simulink model "StarshipSystemModel"  (R2025b)
settings: Solver=VariableStepAuto  StartTime=0.0  StopTime=10.0  RelTol=1e-3
model workspace (MAT data in the model file):
  ActiveGNCMode : Simulink.Bus (value not decoded)
  AerodynamicControlCommand : Simulink.Bus (value not decoded)
  AerodynamicLoad : Simulink.Bus (value not decoded)
  AggregatedStream : Simulink.Bus (value not decoded)
  AllocatedEffectorDemand : Simulink.Bus (value not decoded)
  AttitudeControlDemand : Simulink.Bus (value not decoded)
  AttitudeGuidanceCommand : Simulink.Bus (value not decoded)
  AttitudeRateState : Simulink.Bus (value not decoded)
  AutogenousPressurantGas : Simulink.ConnectionBus (value not decoded)
  CandidateFaultIndication : Simulink.Bus (value not decoded)
  CombustionGasFeed : Simulink.ConnectionBus (value not decoded)
  CommandPathHealth : Simulink.Bus (value not decoded)
  ControlMode : Simulink.ValueType (value not decoded)
  DownlinkSignal : Simulink.Bus (value not decoded)
  ElectricalPower : Simulink.ConnectionBus (value not decoded)
  EngineTelemetry : Simulink.Bus (value not decoded)
  ExecutionContext : Simulink.Bus (value not decoded)
  FaultDiagnosisResult : Simulink.Bus (value not decoded)
  GNCDataContext : Simulink.Bus (value not decoded)
  GNCHealthState : Simulink.Bus (value not decoded)
  GNCStateEstimate : Simulink.Bus (value not decoded)
  GimbalAngle : Simulink.ValueType (value not decoded)
  GimbalMotion : Simulink.ConnectionBus (value not decoded)
  GroundCheckoutLink : Simulink.Bus (value not decoded)
  GroundPressurantSupply : Simulink.ConnectionBus (value not decoded)
  GuidanceConstraints : Simulink.Bus (value not decoded)
  GuidanceMode : Simulink.ValueType (value not decoded)
  LinkHealth : Simulink.Bus (value not decoded)
  LiquidPropellantFeed : Simulink.ConnectionBus (value not decoded)
  MechanicalMotion : Simulink.ConnectionBus (value not decoded)
  MechanismPosition : Simulink.Bus (value not decoded)
  ModeTransitionContext : Simulink.Bus (value not decoded)
  NavigationAidingData : Simulink.Bus (value not decoded)
  NavigationEstimate : Simulink.Bus (value not decoded)
  NavigationHealthStatus : Simulink.Bus (value not decoded)
  NavigationMeasurementSet : Simulink.Bus (value not decoded)
  PercentThrottle : Simulink.ValueType (value not decoded)
  PneumaticActuationGas : Simulink.ConnectionBus (value not decoded)
  PowerConversionStatus : Simulink.Bus (value not decoded)
  PowerDistributionStatus : Simulink.Bus (value not decoded)
  PowerHealthStatus : Simulink.Bus (value not decoded)
  PowerManagementCommand : Simulink.Bus (value not decoded)
  PowerStorageStatus : Simulink.Bus (value not decoded)
  ProtectedThermalState : Simulink.Bus (value not decoded)
  ProtectionIsolationStatus : Simulink.Bus (value not decoded)
  PurgeGasSupply : Simulink.ConnectionBus (value not decoded)
  RCSPulseCommand : Simulink.Bus (value not decoded)
  RCSTelemetry : Simulink.Bus (value not decoded)
  RFFeed : Simulink.ConnectionBus (value not decoded)
  RecoveryMechanismCommand : Simulink.Bus (value not decoded)
  RollThrottleBias : Simulink.ValueType (value not decoded)
  SafetyOverride : Simulink.ValueType (value not decoded)
  SafetyStateStatus : Simulink.Bus (value not decoded)
  ShapedControlDemand : Simulink.Bus (value not decoded)
  SpinStartIgniterGas : Simulink.ConnectionBus (value not decoded)
  StageMechanicalBoundary : Simulink.ConnectionBus (value not decoded)
  StructuralLoad : Simulink.ConnectionBus (value not decoded)
  StructureHealthStatus : Simulink.Bus (value not decoded)
  SubsystemHealthEvidence : Simulink.Bus (value not decoded)
  SubsystemStatusTelemetry : Simulink.Bus (value not decoded)
  TankTelemetry : Simulink.Bus (value not decoded)
  ThermalMonitoringCommand : Simulink.Bus (value not decoded)
  ThermalNetwork : Simulink.ConnectionBus (value not decoded)
  ThrustLoad : Simulink.ConnectionBus (value not decoded)
  TrajectoryGuidanceCommand : Simulink.Bus (value not decoded)
  TrajectoryReference : Simulink.Bus (value not decoded)
  TranslationalControlDemand : Simulink.Bus (value not decoded)
  TranslationalState : Simulink.Bus (value not decoded)
  UplinkSignal : Simulink.Bus (value not decoded)
  ValidatedControlDemand : Simulink.Bus (value not decoded)
  ValveCommand : Simulink.ValueType (value not decoded)
  VehicleStructureState : Simulink.Bus (value not decoded)
  VerifiedCommand : Simulink.Bus (value not decoded)
  VideoStream : Simulink.Bus (value not decoded)
undefined symbols (not defined in the file): ACR, ACT, ASM, ATM, BCR, BDQ, BDR, BDX, BEC, BFC, BHV, BIP, BLM, BNZ, BPI, BPR, BPV, BRX, BSM, BTA, BTP, BVC, BVE, BVV, CAA, CAM, CAS, CAT, CLM, COM, CRS, CTL, CTR, DAQ, ESC, EXT, FCR, FDB, FDE, FEX, FHI, FHM, FIC, FIS, FMG, FSC, GAP, GCM, GMD, GNC, GND, GPH, GTR, HDN, HIA, HSI, IF, INT, LOC, NAI ... (+45)
(part 4 of 8)

== system StarshipSystemModel/Starship/Power & Electrical Energy/Power Management & Monitoring ==
  Bus Element In4 : Inport  PortName=IF-BIP-PIS-01
  Bus Element In2 : Inport  Port=2  PortName=IF-PCM-PSM-01
  Bus Element In1 : Inport  Port=3  PortName=IF-BSM-PSM-01
  Bus Element In3 : Inport  Port=4  PortName=IF-HDN-PSM-01
  Bus Element In5 : Inport  Port=5  PortName=IF-HSI-PIS-01
  Bus Element In6 : Inport  Port=6  PortName=IF-BPI-PIS-01
  Power Management Coordinator : Subsystem
      settings: PortSchema="{\"entries\":[{\"content\":{\"headerSize\":26,\"margin\":15,\"minimumSpacing\":25,\"sides\":[{\"content\":{\"connectorIds\":[\"In1\"]},\"type\":\"ConnectorPlacement.EquallySpacedRectSide\",\"uuid\":\"e231466c-79f3-4a10-9258-08b328dbb315\"},{\"content\":{\"connectorIds\":[\"Out1\",\"Out2\",\"Out3\"],\"side\":\"RIGHT\"},\"type\":\"ConnectorPlacement.EquallySpacedRectSide\",\"uuid\":\"d7277c0a-5b77-426a-ad5b-7f06851f857a\"},{\"content\":{\"side\":\"TOP\"},\"type\":\"ConnectorPlacement.EquallySpacedRectSide\",\"uuid\":\"72d60576-32e4-4fd9-b552-a617024da2ce\"}]},\"type\":\"ConnectorPlacement.EquallySpacedConnector\",\"uuid\":\"6309e805-37c0-4868-97b0-5f8fd0bed587\"}],\"packageUris\":[\"http://schema.mathworks.com/mf0/Connector/R2020b\"],\"version\":\"1.0\"}"
  Power State Monitor : Subsystem
      settings: PortSchema="{\"entries\":[{\"content\":{\"headerSize\":26,\"margin\":15,\"minimumSpacing\":25,\"sides\":[{\"content\":{\"connectorIds\":[\"In2\",\"In3\",\"In1\"]},\"type\":\"ConnectorPlacement.EquallySpacedRectSide\",\"uuid\":\"e231466c-79f3-4a10-9258-08b328dbb315\"},{\"content\":{\"connectorIds\":[\"Out1\"],\"side\":\"RIGHT\"},\"type\":\"ConnectorPlacement.EquallySpacedRectSide\",\"uuid\":\"d7277c0a-5b77-426a-ad5b-7f06851f857a\"},{\"content\":{\"side\":\"TOP\"},\"type\":\"ConnectorPlacement.EquallySpacedRectSide\",\"uuid\":\"72d60576-32e4-4fd9-b552-a617024da2ce\"},{\"content\":{\"side\":\"BOTTOM\"},\"type\":\"ConnectorPlacement.EquallySpacedRectSide\",\"uuid\":\"b6db3a75-7a81-4eda-8d8a-fe1c64e0826f\"}]},\"type\":\"ConnectorPlacement.EquallySpacedConnector\",\"uuid\":\"6309e805-37c0-4868-97b0-5f8fd0bed587\"}],\"packageUris\":[\"http://schema.mathworks.com/mf0/Connector/R2020b\"],\"version\":\"1.0\"}"
  Protection / Isolation Status : Subsystem
      settings: PortSchema="{\"entries\":[{\"content\":{\"headerSize\":26,\"margin\":15,\"minimumSpacing\":25,\"sides\":[{\"content\":{\"connectorIds\":[\"In1\",\"In2\",\"In3\"]},\"type\":\"ConnectorPlacement.EquallySpacedRectSide\",\"uuid\":\"e231466c-79f3-4a10-9258-08b328dbb315\"},{\"content\":{\"side\":\"RIGHT\"},\"type\":\"ConnectorPlacement.EquallySpacedRectSide\",\"uuid\":\"d7277c0a-5b77-426a-ad5b-7f06851f857a\"},{\"content\":{\"side\":\"TOP\"},\"type\":\"ConnectorPlacement.EquallySpacedRectSide\",\"uuid\":\"72d60576-32e4-4fd9-b552-a617024da2ce\"}]},\"type\":\"ConnectorPlacement.EquallySpacedConnector\",\"uuid\":\"6309e805-37c0-4868-97b0-5f8fd0bed587\"}],\"packageUris\":[\"http://schema.mathworks.com/mf0/Connector/R2020b\"],\"version\":\"1.0\"}"
  Bus Element Out1 : Outport  PortName=IF-PMC-BIP-01
  Bus Element Out2 : Outport  Port=2  PortName=IF-PMC-HSI-01
  Bus Element Out3 : Outport  Port=3  PortName=IF-PMM-SAF-01
  wires:
  Bus Element In3/1 -> Power State Monitor/1(IF-HDN-PSM-01)
  Bus Element In5/1 -> Protection / Isolation Status/2(IF-HSI-PIS-01)
  Bus Element In1/1 -> Power State Monitor/3(IF-BSM-PSM-01)
  Bus Element In6/1 -> Protection / Isolation Status/3(IF-BPI-PIS-01)
  Bus Element In2/1 -> Power State Monitor/2(IF-PCM-PSM-01)
  Bus Element In4/1 -> Protection / Isolation Status/1(IF-BIP-PIS-01)
  Power State Monitor/1(IF-PSM-PMC-01) -> Power Management Coordinator/1(IF-PSM-PMC-01)
  Power Management Coordinator/1(IF-PMC-BIP-01) -> Bus Element Out1/1
  Power Management Coordinator/2(IF-PMC-HSI-01) -> Bus Element Out2/1
  Power Management Coordinator/3(IF-PMM-SAF-01) -> Bus Element Out3/1

== system StarshipSystemModel/Starship/Propellent system/Booster propellant System ==
  Bus Element In1 : Inport  PortName=IF-GNC-BFC-01
  Bus Element In2 : Inport  Port=2  PortName=IF-GNC-BPR-01
  Booster propellant tanks : Subsystem
      settings: PortSchema="{\"entries\":[{\"content\":{\"headerSize\":26,\"margin\":15,\"minimumSpacing\":25,\"sides\":[{\"content\":{\"connectorIds\":[\"LConn2\",\"LConn3\",\"LConn4\",\"LConn5\"]},\"type\":\"ConnectorPlacement.EquallySpacedRectSide\",\"uuid\":\"fbe4f8e6-132c-4a0c-8c4c-52d0209da778\"},{\"content\":{\"connectorIds\":[\"LConn1\",\"RConn1\",\"RConn2\",\"RConn3\",\"RConn4\",\"RConn5\"],\"side\":\"RIGHT\"},\"type\":\"ConnectorPlacement.EquallySpacedRectSide\",\"uuid\":\"bbe80fa3-b8e3-44c5-9574-5758a55378fd\"},{\"content\":{\"side\":\"TOP\"},\"type\":\"ConnectorPlacement.EquallySpacedRectSide\",\"uuid\":\"410005e2-e10b-4d3e-a617-d51b1ea5de7e\"}]},\"type\":\"ConnectorPlacement.EquallySpacedConnector\",\"uuid\":\"b66a347a-e5b4-46b1-8a3f-28cf70f30a27\"}],\"packageUris\":[\"http://schema.mathworks.com/mf0/Connector/R2020b\"],\"version\":\"1.0\"}"
  Feed & distribution : Subsystem
      settings: PortSchema="{\"entries\":[{\"content\":{\"headerSize\":26,\"margin\":15,\"minimumSpacing\":25,\"sides\":[{\"content\":{\"connectorIds\":[\"LConn1\",\"LConn2\",\"LConn3\",\"LConn4\",\"LConn5\",\"In1\",\"LConn6\"]},\"type\":\"ConnectorPlacement.EquallySpacedRectSide\",\"uuid\":\"fbe4f8e6-132c-4a0c-8c4c-52d0209da778\"},{\"content\":{\"connectorIds\":[\"RConn1\"],\"side\":\"RIGHT\"},\"type\":\"ConnectorPlacement.EquallySpacedRectSide\",\"uuid\":\"bbe80fa3-b8e3-44c5-9574-5758a55378fd\"},{\"content\":{\"side\":\"TOP\"},\"type\":\"ConnectorPlacement.EquallySpacedRectSide\",\"uuid\":\"410005e2-e10b-4d3e-a617-d51b1ea5de7e\"}]},\"type\":\"ConnectorPlacement.EquallySpacedConnector\",\"uuid\":\"b66a347a-e5b4-46b1-8a3f-28cf70f30a27\"}],\"packageUris\":[\"http://schema.mathworks.com/mf0/Connector/R2020b\"],\"version\":\"1.0\"}"
  Ground propellant interface : Subsystem
      settings: PortSchema="{\"entries\":[{\"content\":{\"headerSize\":26,\"margin\":15,\"minimumSpacing\":25,\"sides\":[{\"content\":{\"connectorIds\":[\"LConn1\",\"LConn2\",\"LConn3\"]},\"type\":\"ConnectorPlacement.EquallySpacedRectSide\",\"uuid\":\"fbe4f8e6-132c-4a0c-8c4c-52d0209da778\"},{\"content\":{\"connectorIds\":[\"RConn1\",\"RConn5\",\"RConn3\",\"RConn2\",\"RConn4\"],\"side\":\"RIGHT\"},\"type\":\"ConnectorPlacement.EquallySpacedRectSide\",\"uuid\":\"bbe80fa3-b8e3-44c5-9574-5758a55378fd\"},{\"content\":{\"side\":\"TOP\"},\"type\":\"ConnectorPlacement.EquallySpacedRectSide\",\"uuid\":\"410005e2-e10b-4d3e-a617-d51b1ea5de7e\"}]},\"type\":\"ConnectorPlacement.EquallySpacedConnector\",\"uuid\":\"b66a347a-e5b4-46b1-8a3f-28cf70f30a27\"}],\"packageUris\":[\"http://schema.mathworks.com/mf0/Connector/R2020b\"],\"version\":\"1.0\"}"
  "Pressurization, purge & venting" : Subsystem
      settings: PortSchema="{\"entries\":[{\"content\":{\"headerSize\":26,\"margin\":15,\"minimumSpacing\":25,\"sides\":[{\"content\":{\"connectorIds\":[\"LConn1\",\"LConn2\",\"LConn3\",\"LConn4\",\"LConn5\",\"LConn6\",\"In1\",\"LConn7\"]},\"type\":\"ConnectorPlacement.EquallySpacedRectSide\",\"uuid\":\"fbe4f8e6-132c-4a0c-8c4c-52d0209da778\"},{\"content\":{\"connectorIds\":[\"RConn1\",\"Out1\",\"RConn2\",\"RConn3\",\"RConn4\",\"RConn5\",\"Out2\",\"RConn6\"],\"side\":\"RIGHT\"},\"type\":\"ConnectorPlacement.EquallySpacedRectSide\",\"uuid\":\"bbe80fa3-b8e3-44c5-9574-5758a55378fd\"},{\"content\":{\"side\":\"TOP\"},\"type\":\"ConnectorPlacement.EquallySpacedRectSide\",\"uuid\":\"410005e2-e10b-4d3e-a617-d51b1ea5de7e\"}]},\"type\":\"ConnectorPlacement.EquallySpacedConnector\",\"uuid\":\"b66a347a-e5b4-46b1-8a3f-28cf70f30a27\"}],\"packageUris\":[\"http://schema.mathworks.com/mf0/Connector/R2020b\"],\"version\":\"1.0\"}"
  IF-BDM-BTP-01 : PMIOPort  Side=Right  ConnectionType=Bus: LiquidPropellantFeed
  IF-BSG-BIG-01 : PMIOPort  Port=2  Side=Right  ConnectionType=Bus: SpinStartIgniterGas
  IF-BNG-BVC-01 : PMIOPort  Port=3  Side=Right  ConnectionType=Bus: PneumaticActuationGas
  IF-BOT-PRS-01 : PMIOPort  Port=4  Side=Left  ConnectionType=Bus: StructuralLoad
  IF-BTP-BPR-01 : PMIOPort  Port=5  Side=Left  ConnectionType=Bus: AutogenousPressurantGas
  "IF-GND-BLQ-01\t" : PMIOPort  Port=6  Side=Left
  "IF-GND-BCQ-01\t" : PMIOPort  Port=7  Side=Left
  IF-PWR-BFC-01 : PMIOPort  Port=8  Side=Left  ConnectionType=Bus: ElectricalPower
  IF-PWR-BPR-01 : PMIOPort  Port=9  Side=Left  ConnectionType=Bus: ElectricalPower
  IF-GND-BPQ-01 : PMIOPort  Port=10  Side=Left  ConnectionType=Bus: GroundPressurantSupply
  Bus Element Out1 : Outport  PortName=IF-BPR-SAF-01
  Bus Element Out2 : Outport  Port=2  PortName=IF-BPR-BTA-01
  wires:
  Bus Element In2/1 -> "Pressurization, purge & venting"/1(IF-GNC-BPR-01)
  "Pressurization, purge & venting"/2(IF-BPR-SAF-01) -> Bus Element Out1/1
  "Pressurization, purge & venting"/1(IF-BPR-BTA-01) -> Bus Element Out2/1
  Bus Element In1/1 -> Feed & distribution/1(IF-GNC-BFC-01)
  connections:
  "IF-GND-BCQ-01\t"/RConn1 -- Ground propellant interface/LConn2
  IF-GND-BPQ-01/RConn1 -- Ground propellant interface/LConn3
  "IF-GND-BLQ-01\t"/RConn1 -- Ground propellant interface/LConn1
  Ground propellant interface/RConn2 -- "Pressurization, purge & venting"/LConn3
  Ground propellant interface/RConn3 -- "Pressurization, purge & venting"/LConn2
  Ground propellant interface/RConn1 -- Booster propellant tanks/LConn2
  Ground propellant interface/RConn5 -- Booster propellant tanks/LConn4
  Ground propellant interface/RConn4 -- "Pressurization, purge & venting"/LConn1
  IF-BTP-BPR-01/RConn1 -- "Pressurization, purge & venting"/LConn4
  "Pressurization, purge & venting"/RConn1 -- IF-BSG-BIG-01/RConn1
  Feed & distribution/RConn1 -- IF-BDM-BTP-01/RConn1
  "Pressurization, purge & venting"/RConn2 -- Booster propellant tanks/LConn5
  "Pressurization, purge & venting"/RConn3 -- Feed & distribution/LConn3
  "Pressurization, purge & venting"/RConn4 -- Feed & distribution/LConn4
  "Pressurization, purge & venting"/RConn5 -- Booster propellant tanks/LConn3
  "Pressurization, purge & venting"/RConn6 -- IF-BNG-BVC-01/RConn1
  Booster propellant tanks/RConn5 -- Feed & distribution/LConn2
  Booster propellant tanks/RConn1 -- Feed & distribution/LConn1
  Booster propellant tanks/RConn2 -- Feed & distribution/LConn5
  Booster propellant tanks/RConn3 -- "Pressurization, purge & venting"/LConn6
  Booster propellant tanks/RConn4 -- "Pressurization, purge & venting"/LConn5
  IF-BOT-PRS-01/RConn1 -- Booster propellant tanks/LConn1
  IF-PWR-BFC-01/RConn1 -- Feed & distribution/LConn6
  IF-PWR-BPR-01/RConn1 -- "Pressurization, purge & venting"/LConn7

== system StarshipSystemModel/Starship/Propellent system/Ship propellant System ==
  Bus Element In1 : Inport  PortName=IF-GNC-SFC-01
  Bus Element In2 : Inport  Port=2  PortName=IF-GNC-SPR-01
  Feed & distribution : Subsystem
      settings: PortSchema="{\"entries\":[{\"content\":{\"headerSize\":26,\"margin\":15,\"minimumSpacing\":25,\"sides\":[{\"content\":{\"connectorIds\":[\"LConn1\",\"In1\",\"LConn2\",\"LConn3\",\"LConn4\",\"LConn5\",\"LConn6\",\"LConn7\"]},\"type\":\"ConnectorPlacement.EquallySpacedRectSide\",\"uuid\":\"fbe4f8e6-132c-4a0c-8c4c-52d0209da778\"},{\"content\":{\"connectorIds\":[\"RConn1\"],\"side\":\"RIGHT\"},\"type\":\"ConnectorPlacement.EquallySpacedRectSide\",\"uuid\":\"bbe80fa3-b8e3-44c5-9574-5758a55378fd\"},{\"content\":{\"side\":\"TOP\"},\"type\":\"ConnectorPlacement.EquallySpacedRectSide\",\"uuid\":\"410005e2-e10b-4d3e-a617-d51b1ea5de7e\"}]},\"type\":\"ConnectorPlacement.EquallySpacedConnector\",\"uuid\":\"b66a347a-e5b4-46b1-8a3f-28cf70f30a27\"}],\"packageUris\":[\"http://schema.mathworks.com/mf0/Connector/R2020b\"],\"version\":\"1.0\"}"
  Ground propellant interface : Subsystem
      settings: PortSchema="{\"entries\":[{\"content\":{\"headerSize\":26,\"margin\":15,\"minimumSpacing\":25,\"sides\":[{\"content\":{\"connectorIds\":[\"LConn1\",\"LConn2\",\"LConn3\"]},\"type\":\"ConnectorPlacement.EquallySpacedRectSide\",\"uuid\":\"fbe4f8e6-132c-4a0c-8c4c-52d0209da778\"},{\"content\":{\"connectorIds\":[\"RConn1\",\"RConn2\",\"RConn3\",\"RConn4\",\"RConn5\"],\"side\":\"RIGHT\"},\"type\":\"ConnectorPlacement.EquallySpacedRectSide\",\"uuid\":\"bbe80fa3-b8e3-44c5-9574-5758a55378fd\"},{\"content\":{\"side\":\"TOP\"},\"type\":\"ConnectorPlacement.EquallySpacedRectSide\",\"uuid\":\"410005e2-e10b-4d3e-a617-d51b1ea5de7e\"}]},\"type\":\"ConnectorPlacement.EquallySpacedConnector\",\"uuid\":\"b66a347a-e5b4-46b1-8a3f-28cf70f30a27\"}],\"packageUris\":[\"http://schema.mathworks.com/mf0/Connector/R2020b\"],\"version\":\"1.0\"}"
  "Pressurization, purge & venting" : Subsystem
      settings: PortSchema="{\"entries\":[{\"content\":{\"headerSize\":26,\"margin\":15,\"minimumSpacing\":25,\"sides\":[{\"content\":{\"connectorIds\":[\"LConn1\",\"LConn2\",\"LConn3\",\"LConn4\",\"LConn5\",\"LConn6\",\"In1\",\"LConn7\"]},\"type\":\"ConnectorPlacement.EquallySpacedRectSide\",\"uuid\":\"fbe4f8e6-132c-4a0c-8c4c-52d0209da778\"},{\"content\":{\"connectorIds\":[\"RConn1\",\"Out1\",\"RConn2\",\"RConn3\",\"RConn4\",\"RConn5\",\"Out2\",\"RConn6\",\"RConn7\"],\"side\":\"RIGHT\"},\"type\":\"ConnectorPlacement.EquallySpacedRectSide\",\"uuid\":\"bbe80fa3-b8e3-44c5-9574-5758a55378fd\"},{\"content\":{\"side\":\"TOP\"},\"type\":\"ConnectorPlacement.EquallySpacedRectSide\",\"uuid\":\"410005e2-e10b-4d3e-a617-d51b1ea5de7e\"}]},\"type\":\"ConnectorPlacement.EquallySpacedConnector\",\"uuid\":\"b66a347a-e5b4-46b1-8a3f-28cf70f30a27\"}],\"packageUris\":[\"http://schema.mathworks.com/mf0/Connector/R2020b\"],\"version\":\"1.0\"}"
  Ship propellant tanks : Subsystem
      settings: PortSchema="{\"entries\":[{\"content\":{\"headerSize\":26,\"margin\":15,\"minimumSpacing\":25,\"sides\":[{\"content\":{\"connectorIds\":[\"LConn2\",\"LConn3\",\"LConn4\",\"LConn5\"]},\"type\":\"ConnectorPlacement.EquallySpacedRectSide\",\"uuid\":\"fbe4f8e6-132c-4a0c-8c4c-52d0209da778\"},{\"content\":{\"connectorIds\":[\"LConn1\",\"RConn4\",\"RConn1\",\"RConn3\",\"RConn2\",\"RConn5\",\"RConn6\"],\"side\":\"RIGHT\"},\"type\":\"ConnectorPlacement.EquallySpacedRectSide\",\"uuid\":\"bbe80fa3-b8e3-44c5-9574-5758a55378fd\"},{\"content\":{\"side\":\"TOP\"},\"type\":\"ConnectorPlacement.EquallySpacedRectSide\",\"uuid\":\"410005e2-e10b-4d3e-a617-d51b1ea5de7e\"}]},\"type\":\"ConnectorPlacement.EquallySpacedConnector\",\"uuid\":\"b66a347a-e5b4-46b1-8a3f-28cf70f30a27\"}],\"packageUris\":[\"http://schema.mathworks.com/mf0/Connector/R2020b\"],\"version\":\"1.0\"}"
  IF-PWR-SPR-01 : PMIOPort  Side=Right  ConnectionType=Bus: ElectricalPower
  IF-SSG-SIG-01 : PMIOPort  Port=2  Side=Right  ConnectionType=Bus: SpinStartIgniterGas
  IF-SNG-SVC-01 : PMIOPort  Port=3  Side=Right  ConnectionType=Bus: PneumaticActuationGas
  IF-SPR-RVM-01 : PMIOPort  Port=4  Side=Right  ConnectionType=Bus: CombustionGasFeed
  IF-SDM-STP-01 : PMIOPort  Port=5  Side=Right  ConnectionType=Bus: LiquidPropellantFeed
  IF-SOT-PRS-01 : PMIOPort  Port=6  Side=Left  ConnectionType=Bus: StructuralLoad
  IF-STP-SPR-01 : PMIOPort  Port=7  Side=Left  ConnectionType=Bus: AutogenousPressurantGas
  IF-GND-SLQ-01 : PMIOPort  Port=8  Side=Left
  IF-GND-SCQ-01 : PMIOPort  Port=9  Side=Left
  IF-PWR-SFC-01 : PMIOPort  Port=10  Side=Left  ConnectionType=Bus: ElectricalPower
  IF-GND-SPQ-01 : PMIOPort  Port=11  Side=Left  ConnectionType=Bus: GroundPressurantSupply
  Bus Element Out1 : Outport  PortName=IF-SPR-SAF-01
  Bus Element Out2 : Outport  Port=2  PortName=IF-SPR-STA-01
  wires:
  Bus Element In2/1 -> "Pressurization, purge & venting"/1(IF-GNC-SPR-01)
  Bus Element In1/1 -> Feed & distribution/1(IF-GNC-SFC-01)
  "Pressurization, purge & venting"/2(IF-SPR-STA-01) -> Bus Element Out2/1
  "Pressurization, purge & venting"/1(IF-SPR-SAF-01) -> Bus Element Out1/1
  connections:
  IF-GND-SPQ-01/RConn1 -- Ground propellant interface/LConn3
  IF-GND-SCQ-01/RConn1 -- Ground propellant interface/LConn2
  IF-GND-SLQ-01/RConn1 -- Ground propellant interface/LConn1
  Ground propellant interface/RConn5 -- Ship propellant tanks/LConn4
  Ground propellant interface/RConn4 -- "Pressurization, purge & venting"/LConn6
  Ground propellant interface/RConn3 -- "Pressurization, purge & venting"/LConn5
  Ground propellant interface/RConn2 -- "Pressurization, purge & venting"/LConn4
  Ground propellant interface/RConn1 -- Ship propellant tanks/LConn5
  IF-STP-SPR-01/RConn1 -- "Pressurization, purge & venting"/LConn1
  Ship propellant tanks/RConn4 -- "Pressurization, purge & venting"/LConn2
  "Pressurization, purge & venting"/RConn4 -- Feed & distribution/LConn1
  Ship propellant tanks/RConn1 -- Feed & distribution/LConn2
  "Pressurization, purge & venting"/RConn7 -- IF-SPR-RVM-01/RConn1
  Ship propellant tanks/RConn3 -- "Pressurization, purge & venting"/LConn3
  Ship propellant tanks/RConn2 -- Feed & distribution/LConn3
  "Pressurization, purge & venting"/RConn2 -- Ship propellant tanks/LConn3
  Ship propellant tanks/RConn5 -- Feed & distribution/LConn4
  Ship propellant tanks/RConn6 -- Feed & distribution/LConn5
  "Pressurization, purge & venting"/RConn5 -- Feed & distribution/LConn6
  "Pressurization, purge & venting"/RConn1 -- IF-SSG-SIG-01/RConn1
  "Pressurization, purge & venting"/RConn3 -- Ship propellant tanks/LConn2
  "Pressurization, purge & venting"/RConn6 -- IF-SNG-SVC-01/RConn1
  Feed & distribution/RConn1 -- IF-SDM-STP-01/RConn1
  IF-SOT-PRS-01/RConn1 -- Ship propellant tanks/LConn1
  IF-PWR-SFC-01/RConn1 -- Feed & distribution/LConn7
  IF-PWR-SPR-01/RConn1 -- "Pressurization, purge & venting"/LConn7

== system StarshipSystemModel/Starship/Propulsion/Booster main engines ==
  Bus Element In1 : Inport  PortName=IF-GNC-BEC-01
  Bus Element In2 : Inport  Port=2  PortName=IF-SAF-BEC-01
  "Combustion Chamber " : Subsystem
      settings: PortSchema="{\"entries\":[{\"content\":{\"headerSize\":26,\"margin\":15,\"minimumSpacing\":25,\"sides\":[{\"content\":{\"connectorIds\":[\"LConn1\"]},\"type\":\"ConnectorPlacement.EquallySpacedRectSide\",\"uuid\":\"315fc4b8-96c1-4575-a6b3-eadee3c565c5\"},{\"content\":{\"connectorIds\":[\"RConn1\"],\"side\":\"RIGHT\"},\"type\":\"ConnectorPlacement.EquallySpacedRectSide\",\"uuid\":\"3e876d4b-731c-46c4-97d4-16d95cf44eb6\"},{\"content\":{\"side\":\"TOP\"},\"type\":\"ConnectorPlacement.EquallySpacedRectSide\",\"uuid\":\"b527a8d5-4fb1-4a9d-8105-fff73624f75e\"}]},\"type\":\"ConnectorPlacement.EquallySpacedConnector\",\"uuid\":\"4da3c338-7f32-408f-a75b-02b41c006a8f\"}],\"packageUris\":[\"http://schema.mathworks.com/mf0/Connector/R2020b\"],\"version\":\"1.0\"}"
  Engine controller : Subsystem
      settings: PortSchema="{\"entries\":[{\"content\":{\"headerSize\":26,\"margin\":15,\"minimumSpacing\":25,\"sides\":[{\"content\":{\"connectorIds\":[\"LConn1\",\"In1\",\"In2\"]},\"type\":\"ConnectorPlacement.EquallySpacedRectSide\",\"uuid\":\"a24f90f9-b52e-4407-98a2-61cef3ed1001\"},{\"content\":{\"connectorIds\":[\"Out1\",\"Out2\",\"Out3\"],\"side\":\"RIGHT\"},\"type\":\"ConnectorPlacement.EquallySpacedRectSide\",\"uuid\":\"349c89d4-9966-4ad9-ba76-db4d38641e72\"},{\"content\":{\"side\":\"TOP\"},\"type\":\"ConnectorPlacement.EquallySpacedRectSide\",\"uuid\":\"c23b8a3e-5693-4bb4-96b3-90d999333c4e\"}]},\"type\":\"ConnectorPlacement.EquallySpacedConnector\",\"uuid\":\"ab682651-c32f-4460-8c4f-01dcf64563ad\"}],\"packageUris\":[\"http://schema.mathworks.com/mf0/Connector/R2020b\"],\"version\":\"1.0\"}"
  Ignition system : Subsystem
      settings: PortSchema="{\"entries\":[{\"content\":{\"headerSize\":26,\"margin\":15,\"minimumSpacing\":25,\"sides\":[{\"content\":{\"connectorIds\":[\"LConn1\"]},\"type\":\"ConnectorPlacement.EquallySpacedRectSide\",\"uuid\":\"a24f90f9-b52e-4407-98a2-61cef3ed1001\"},{\"content\":{\"connectorIds\":[\"RConn1\"],\"side\":\"RIGHT\"},\"type\":\"ConnectorPlacement.EquallySpacedRectSide\",\"uuid\":\"349c89d4-9966-4ad9-ba76-db4d38641e72\"},{\"content\":{\"side\":\"TOP\"},\"type\":\"ConnectorPlacement.EquallySpacedRectSide\",\"uuid\":\"c23b8a3e-5693-4bb4-96b3-90d999333c4e\"}]},\"type\":\"ConnectorPlacement.EquallySpacedConnector\",\"uuid\":\"ab682651-c32f-4460-8c4f-01dcf64563ad\"}],\"packageUris\":[\"http://schema.mathworks.com/mf0/Connector/R2020b\"],\"version\":\"1.0\"}"
  Mounting interface : Subsystem
      settings: PortSchema="{\"entries\":[{\"content\":{\"headerSize\":26,\"margin\":15,\"minimumSpacing\":25,\"sides\":[{\"content\":{\"connectorIds\":[\"LConn1\"]},\"type\":\"ConnectorPlacement.EquallySpacedRectSide\",\"uuid\":\"a24f90f9-b52e-4407-98a2-61cef3ed1001\"},{\"content\":{\"connectorIds\":[\"RConn1\"],\"side\":\"RIGHT\"},\"type\":\"ConnectorPlacement.EquallySpacedRectSide\",\"uuid\":\"349c89d4-9966-4ad9-ba76-db4d38641e72\"},{\"content\":{\"side\":\"TOP\"},\"type\":\"ConnectorPlacement.EquallySpacedRectSide\",\"uuid\":\"c23b8a3e-5693-4bb4-96b3-90d999333c4e\"}]},\"type\":\"ConnectorPlacement.EquallySpacedConnector\",\"uuid\":\"ab682651-c32f-4460-8c4f-01dcf64563ad\"}],\"packageUris\":[\"http://schema.mathworks.com/mf0/Connector/R2020b\"],\"version\":\"1.0\"}"
  Nozzle : Subsystem
      settings: PortSchema="{\"entries\":[{\"content\":{\"headerSize\":26,\"margin\":15,\"minimumSpacing\":25,\"sides\":[{\"content\":{\"connectorIds\":[\"LConn1\"]},\"type\":\"ConnectorPlacement.EquallySpacedRectSide\",\"uuid\":\"315fc4b8-96c1-4575-a6b3-eadee3c565c5\"},{\"content\":{\"connectorIds\":[\"Out1\"],\"side\":\"RIGHT\"},\"type\":\"ConnectorPlacement.EquallySpacedRectSide\",\"uuid\":\"3e876d4b-731c-46c4-97d4-16d95cf44eb6\"},{\"content\":{\"side\":\"TOP\"},\"type\":\"ConnectorPlacement.EquallySpacedRectSide\",\"uuid\":\"b527a8d5-4fb1-4a9d-8105-fff73624f75e\"}]},\"type\":\"ConnectorPlacement.EquallySpacedConnector\",\"uuid\":\"4da3c338-7f32-408f-a75b-02b41c006a8f\"}],\"packageUris\":[\"http://schema.mathworks.com/mf0/Connector/R2020b\"],\"version\":\"1.0\"}"
  Preburners : Subsystem
      settings: PortSchema="{\"entries\":[{\"content\":{\"headerSize\":26,\"margin\":15,\"minimumSpacing\":25,\"sides\":[{\"content\":{\"connectorIds\":[\"LConn1\",\"LConn2\"]},\"type\":\"ConnectorPlacement.EquallySpacedRectSide\",\"uuid\":\"315fc4b8-96c1-4575-a6b3-eadee3c565c5\"},{\"content\":{\"connectorIds\":[\"RConn1\"],\"side\":\"RIGHT\"},\"type\":\"ConnectorPlacement.EquallySpacedRectSide\",\"uuid\":\"3e876d4b-731c-46c4-97d4-16d95cf44eb6\"},{\"content\":{\"side\":\"TOP\"},\"type\":\"ConnectorPlacement.EquallySpacedRectSide\",\"uuid\":\"b527a8d5-4fb1-4a9d-8105-fff73624f75e\"}]},\"type\":\"ConnectorPlacement.EquallySpacedConnector\",\"uuid\":\"4da3c338-7f32-408f-a75b-02b41c006a8f\"}],\"packageUris\":[\"http://schema.mathworks.com/mf0/Connector/R2020b\"],\"version\":\"1.0\"}"
  Turbopumps : Subsystem
      settings: PortSchema="{\"entries\":[{\"content\":{\"headerSize\":26,\"margin\":15,\"minimumSpacing\":25,\"sides\":[{\"content\":{\"connectorIds\":[\"LConn1\",\"LConn2\"]},\"type\":\"ConnectorPlacement.EquallySpacedRectSide\",\"uuid\":\"315fc4b8-96c1-4575-a6b3-eadee3c565c5\"},{\"content\":{\"connectorIds\":[\"RConn1\",\"RConn2\"],\"side\":\"RIGHT\"},\"type\":\"ConnectorPlacement.EquallySpacedRectSide\",\"uuid\":\"3e876d4b-731c-46c4-97d4-16d95cf44eb6\"},{\"content\":{\"side\":\"TOP\"},\"type\":\"ConnectorPlacement.EquallySpacedRectSide\",\"uuid\":\"b527a8d5-4fb1-4a9d-8105-fff73624f75e\"}]},\"type\":\"ConnectorPlacement.EquallySpacedConnector\",\"uuid\":\"4da3c338-7f32-408f-a75b-02b41c006a8f\"}],\"packageUris\":[\"http://schema.mathworks.com/mf0/Connector/R2020b\"],\"version\":\"1.0\"}"
  Valves & control : Subsystem
      settings: PortSchema="{\"entries\":[{\"content\":{\"headerSize\":26,\"margin\":15,\"minimumSpacing\":25,\"sides\":[{\"content\":{\"connectorIds\":[\"In1\",\"LConn1\"]},\"type\":\"ConnectorPlacement.EquallySpacedRectSide\",\"uuid\":\"a24f90f9-b52e-4407-98a2-61cef3ed1001\"},{\"content\":{\"connectorIds\":[\"RConn1\"],\"side\":\"RIGHT\"},\"type\":\"ConnectorPlacement.EquallySpacedRectSide\",\"uuid\":\"349c89d4-9966-4ad9-ba76-db4d38641e72\"},{\"content\":{\"side\":\"TOP\"},\"type\":\"ConnectorPlacement.EquallySpacedRectSide\",\"uuid\":\"c23b8a3e-5693-4bb4-96b3-90d999333c4e\"}]},\"type\":\"ConnectorPlacement.EquallySpacedConnector\",\"uuid\":\"ab682651-c32f-4460-8c4f-01dcf64563ad\"}],\"packageUris\":[\"http://schema.mathworks.com/mf0/Connector/R2020b\"],\"version\":\"1.0\"}"
  IF-PWR-BEC-01 : PMIOPort  Side=Left  ConnectionType=Bus: ElectricalPower
  IF-BMT-TLI-01 : PMIOPort  Port=2  Side=Left  ConnectionType=Bus: StructuralLoad
  IF-BDM-BTP-01 : PMIOPort  Port=3  Side=Left  ConnectionType=Bus: LiquidPropellantFeed
  IF-BTP-BPR-01 : PMIOPort  Port=4  Side=Right  ConnectionType=Bus: AutogenousPressurantGas
  IF-BSG-BIG-01 : PMIOPort  Port=5  Side=Left  ConnectionType=Bus: SpinStartIgniterGas
  IF-BNG-BVC-01 : PMIOPort  Port=6  Side=Left  ConnectionType=Bus: PneumaticActuationGas
  IF-GMB-BMT-01 : PMIOPort  Port=7  Side=Left  ConnectionType=Bus: GimbalMotion
  Bus Element Out1 : Outport  PortName=IF-BEC-SAF-01
  Bus Element Out2 : Outport  Port=2  PortName=IF-BEC-BTA-01
  Bus Element Out3 : Outport  Port=3  PortName=IF-BNZ-BTP-01
  wires:
  Bus Element In2/1 -> Engine controller/2(IF-SAF-BEC-01)
  Bus Element In1/1 -> Engine controller/1(IF-GNC-BEC-01)
  Engine controller/2(IF-BEC-BTA-01) -> Bus Element Out2/1
  Engine controller/1(IF-BEC-SAF-01) -> Bus Element Out1/1
  Engine controller/3(IF-BEC-BVC-01) -> Valves & control/1(IF-BEC-BVC-01)
  Nozzle/1(IF-BNZ-BTP-01) -> Bus Element Out3/1
  connections:
  IF-BDM-BTP-01/RConn1 -- Turbopumps/LConn1
  IF-GMB-BMT-01/RConn1 -- Mounting interface/LConn1
  Preburners/RConn1 -- "Combustion Chamber "/LConn1
  Valves & control/RConn1 -- Turbopumps/LConn2
  Turbopumps/RConn2 -- Preburners/LConn1
  Ignition system/RConn1 -- Preburners/LConn2
  "Combustion Chamber "/RConn1 -- Nozzle/LConn1
  IF-BSG-BIG-01/RConn1 -- Ignition system/LConn1
  IF-BNG-BVC-01/RConn1 -- Valves & control/LConn1
  Turbopumps/RConn1 -- IF-BTP-BPR-01/RConn1
  IF-BMT-TLI-01/RConn1 -- Mounting interface/RConn1
  IF-PWR-BEC-01/RConn1 -- Engine controller/LConn1

== system StarshipSystemModel/Starship/Propulsion/Gimbal // TVC actuation ==
  Bus Element In1 : Inport  PortName=IF-GNC-TVC-01
  Gimbal bearing : Subsystem
      settings: PortSchema="{\"entries\":[{\"content\":{\"headerSize\":26,\"margin\":15,\"minimumSpacing\":25,\"sides\":[{\"content\":{\"connectorIds\":[\"LConn1\",\"LConn2\"]},\"type\":\"ConnectorPlacement.EquallySpacedRectSide\",\"uuid\":\"a24f90f9-b52e-4407-98a2-61cef3ed1001\"},{\"content\":{\"connectorIds\":[\"RConn1\",\"RConn2\"],\"side\":\"RIGHT\"},\"type\":\"ConnectorPlacement.EquallySpacedRectSide\",\"uuid\":\"349c89d4-9966-4ad9-ba76-db4d38641e72\"},{\"content\":{\"side\":\"TOP\"},\"type\":\"ConnectorPlacement.EquallySpacedRectSide\",\"uuid\":\"c23b8a3e-5693-4bb4-96b3-90d999333c4e\"}]},\"type\":\"ConnectorPlacement.EquallySpacedConnector\",\"uuid\":\"ab682651-c32f-4460-8c4f-01dcf64563ad\"}],\"packageUris\":[\"http://schema.mathworks.com/mf0/Connector/R2020b\"],\"version\":\"1.0\"}"
  Pitch actuator : Subsystem
      settings: PortSchema="{\"entries\":[{\"content\":{\"headerSize\":26,\"margin\":15,\"minimumSpacing\":25,\"sides\":[{\"content\":{\"connectorIds\":[\"In1\"]},\"type\":\"ConnectorPlacement.EquallySpacedRectSide\",\"uuid\":\"a24f90f9-b52e-4407-98a2-61cef3ed1001\"},{\"content\":{\"connectorIds\":[\"RConn1\"],\"side\":\"RIGHT\"},\"type\":\"ConnectorPlacement.EquallySpacedRectSide\",\"uuid\":\"349c89d4-9966-4ad9-ba76-db4d38641e72\"},{\"content\":{\"side\":\"TOP\"},\"type\":\"ConnectorPlacement.EquallySpacedRectSide\",\"uuid\":\"c23b8a3e-5693-4bb4-96b3-90d999333c4e\"},{\"content\":{\"side\":\"BOTTOM\"},\"type\":\"ConnectorPlacement.EquallySpacedRectSide\",\"uuid\":\"53421d2e-cd64-4a64-9551-ba2d9208335d\"}]},\"type\":\"ConnectorPlacement.EquallySpacedConnector\",\"uuid\":\"ab682651-c32f-4460-8c4f-01dcf64563ad\"}],\"packageUris\":[\"http://schema.mathworks.com/mf0/Connector/R2020b\"],\"version\":\"1.0\"}"
  TVC controller : Subsystem
      settings: PortSchema="{\"entries\":[{\"content\":{\"headerSize\":26,\"margin\":15,\"minimumSpacing\":25,\"sides\":[{\"content\":{\"connectorIds\":[\"LConn1\",\"In1\"]},\"type\":\"ConnectorPlacement.EquallySpacedRectSide\",\"uuid\":\"a24f90f9-b52e-4407-98a2-61cef3ed1001\"},{\"content\":{\"connectorIds\":[\"Out1\",\"Out2\",\"Out3\"],\"side\":\"RIGHT\"},\"type\":\"ConnectorPlacement.EquallySpacedRectSide\",\"uuid\":\"349c89d4-9966-4ad9-ba76-db4d38641e72\"},{\"content\":{\"side\":\"TOP\"},\"type\":\"ConnectorPlacement.EquallySpacedRectSide\",\"uuid\":\"c23b8a3e-5693-4bb4-96b3-90d999333c4e\"}]},\"type\":\"ConnectorPlacement.EquallySpacedConnector\",\"uuid\":\"ab682651-c32f-4460-8c4f-01dcf64563ad\"}],\"packageUris\":[\"http://schema.mathworks.com/mf0/Connector/R2020b\"],\"version\":\"1.0\"}"
  Yaw actuator : Subsystem
      settings: PortSchema="{\"entries\":[{\"content\":{\"headerSize\":26,\"margin\":15,\"minimumSpacing\":25,\"sides\":[{\"content\":{\"connectorIds\":[\"In1\"]},\"type\":\"ConnectorPlacement.EquallySpacedRectSide\",\"uuid\":\"a24f90f9-b52e-4407-98a2-61cef3ed1001\"},{\"content\":{\"connectorIds\":[\"RConn1\"],\"side\":\"RIGHT\"},\"type\":\"ConnectorPlacement.EquallySpacedRectSide\",\"uuid\":\"349c89d4-9966-4ad9-ba76-db4d38641e72\"},{\"content\":{\"side\":\"TOP\"},\"type\":\"ConnectorPlacement.EquallySpacedRectSide\",\"uuid\":\"c23b8a3e-5693-4bb4-96b3-90d999333c4e\"}]},\"type\":\"ConnectorPlacement.EquallySpacedConnector\",\"uuid\":\"ab682651-c32f-4460-8c4f-01dcf64563ad\"}],\"packageUris\":[\"http://schema.mathworks.com/mf0/Connector/R2020b\"],\"version\":\"1.0\"}"
  IF-GMB-BMT-01 : PMIOPort  Side=Right  ConnectionType=Bus: GimbalMotion
  IF-GMB-SMT-01 : PMIOPort  Port=2  Side=Right  ConnectionType=Bus: GimbalMotion
  IF-PWR-TVC-01 : PMIOPort  Port=3  Side=Left  ConnectionType=Bus: ElectricalPower
  Bus Element Out1 : Outport  PortName=IF-TVC-GNC-01
  wires:
  Bus Element In1/1 -> TVC controller/1(IF-GNC-TVC-01)
  TVC controller/1(IF-TVC-GNC-01) -> Bus Element Out1/1
  TVC controller/3(IF-TVC-PAC-01) -> Pitch actuator/1(IF-TVC-PAC-01)
  TVC controller/2(IF-TVC-YAC-01) -> Yaw actuator/1(IF-TVC-YAC-01)
  connections:
  Gimbal bearing/RConn1 -- IF-GMB-BMT-01/RConn1
  Pitch actuator/RConn1 -- Gimbal bearing/LConn2
  Yaw actuator/RConn1 -- Gimbal bearing/LConn1
  Gimbal bearing/RConn2 -- IF-GMB-SMT-01/RConn1
  IF-PWR-TVC-01/RConn1 -- TVC controller/LConn1

== system StarshipSystemModel/Starship/Propulsion/RCS thrusters ==
  Bus Element In1 : Inport  PortName=IF-GNC-RCT-01
  Igniter : Subsystem
      settings: PortSchema="{\"entries\":[{\"content\":{\"headerSize\":26,\"margin\":15,\"minimumSpacing\":25,\"sides\":[{\"content\":{},\"type\":\"ConnectorPlacement.EquallySpacedRectSide\",\"uuid\":\"a24f90f9-b52e-4407-98a2-61cef3ed1001\"},{\"content\":{\"connectorIds\":[\"RConn1\"],\"side\":\"RIGHT\"},\"type\":\"ConnectorPlacement.EquallySpacedRectSide\",\"uuid\":\"349c89d4-9966-4ad9-ba76-db4d38641e72\"},{\"content\":{\"side\":\"TOP\"},\"type\":\"ConnectorPlacement.EquallySpacedRectSide\",\"uuid\":\"c23b8a3e-5693-4bb4-96b3-90d999333c4e\"}]},\"type\":\"ConnectorPlacement.EquallySpacedConnector\",\"uuid\":\"ab682651-c32f-4460-8c4f-01dcf64563ad\"}],\"packageUris\":[\"http://schema.mathworks.com/mf0/Connector/R2020b\"],\"version\":\"1.0\"}"
  RCS controller : Subsystem
      settings: PortSchema="{\"entries\":[{\"content\":{\"headerSize\":26,\"margin\":15,\"minimumSpacing\":25,\"sides\":[{\"content\":{\"connectorIds\":[\"LConn1\",\"In1\"]},\"type\":\"ConnectorPlacement.EquallySpacedRectSide\",\"uuid\":\"a24f90f9-b52e-4407-98a2-61cef3ed1001\"},{\"content\":{\"connectorIds\":[\"Out1\",\"Out2\"],\"side\":\"RIGHT\"},\"type\":\"ConnectorPlacement.EquallySpacedRectSide\",\"uuid\":\"349c89d4-9966-4ad9-ba76-db4d38641e72\"},{\"content\":{\"side\":\"TOP\"},\"type\":\"ConnectorPlacement.EquallySpacedRectSide\",\"uuid\":\"c23b8a3e-5693-4bb4-96b3-90d999333c4e\"}]},\"type\":\"ConnectorPlacement.EquallySpacedConnector\",\"uuid\":\"ab682651-c32f-4460-8c4f-01dcf64563ad\"}],\"packageUris\":[\"http://schema.mathworks.com/mf0/Connector/R2020b\"],\"version\":\"1.0\"}"
  "Thruster chamber, nozzle" : Subsystem
      settings: PortSchema="{\"entries\":[{\"content\":{\"headerSize\":26,\"margin\":15,\"minimumSpacing\":25,\"sides\":[{\"content\":{\"connectorIds\":[\"LConn2\",\"LConn1\"]},\"type\":\"ConnectorPlacement.EquallySpacedRectSide\",\"uuid\":\"a24f90f9-b52e-4407-98a2-61cef3ed1001\"},{\"content\":{\"side\":\"RIGHT\"},\"type\":\"ConnectorPlacement.EquallySpacedRectSide\",\"uuid\":\"349c89d4-9966-4ad9-ba76-db4d38641e72\"},{\"content\":{\"side\":\"TOP\"},\"type\":\"ConnectorPlacement.EquallySpacedRectSide\",\"uuid\":\"c23b8a3e-5693-4bb4-96b3-90d999333c4e\"}]},\"type\":\"ConnectorPlacement.EquallySpacedConnector\",\"uuid\":\"ab682651-c32f-4460-8c4f-01dcf64563ad\"}],\"packageUris\":[\"http://schema.mathworks.com/mf0/Connector/R2020b\"],\"version\":\"1.0\"}"
  Valve & feed manifold : Subsystem
      settings: PortSchema="{\"entries\":[{\"content\":{\"headerSize\":26,\"margin\":15,\"minimumSpacing\":25,\"sides\":[{\"content\":{\"connectorIds\":[\"LConn1\",\"In1\"]},\"type\":\"ConnectorPlacement.EquallySpacedRectSide\",\"uuid\":\"a24f90f9-b52e-4407-98a2-61cef3ed1001\"},{\"content\":{\"connectorIds\":[\"RConn1\"],\"side\":\"RIGHT\"},\"type\":\"ConnectorPlacement.EquallySpacedRectSide\",\"uuid\":\"349c89d4-9966-4ad9-ba76-db4d38641e72\"},{\"content\":{\"side\":\"TOP\"},\"type\":\"ConnectorPlacement.EquallySpacedRectSide\",\"uuid\":\"c23b8a3e-5693-4bb4-96b3-90d999333c4e\"}]},\"type\":\"ConnectorPlacement.EquallySpacedConnector\",\"uuid\":\"ab682651-c32f-4460-8c4f-01dcf64563ad\"}],\"packageUris\":[\"http://schema.mathworks.com/mf0/Connector/R2020b\"],\"version\":\"1.0\"}"
  IF-PWR-RCT-01 : PMIOPort  Side=Left  ConnectionType=Bus: ElectricalPower
  IF-SPR-RVM-01 : PMIOPort  Port=2  Side=Left  ConnectionType=Bus: CombustionGasFeed
  Bus Element Out1 : Outport  PortName=IF-RCT-SAF-01
  wires:
  Bus Element In1/1 -> RCS controller/1(IF-GNC-RCT-01)
  RCS controller/2(IF-RCT-RVM-01) -> Valve & feed manifold/1(IF-RCT-RVM-01)
  RCS controller/1(IF-RCT-SAF-01) -> Bus Element Out1/1
  connections:
  Igniter/RConn1 -- "Thruster chamber, nozzle"/LConn2
  Valve & feed manifold/RConn1 -- "Thruster chamber, nozzle"/LConn1
  IF-SPR-RVM-01/RConn1 -- Valve & feed manifold/LConn1
  IF-PWR-RCT-01/RConn1 -- RCS controller/LConn1

== system StarshipSystemModel/Starship/Propulsion/Ship main engines ==
  Bus Element In1 : Inport  PortName=IF-GNC-SEC-01
  Bus Element In2 : Inport  Port=2  PortName=IF-SAF-SEC-01
  "Combustion Chamber " : Subsystem
      settings: PortSchema="{\"entries\":[{\"content\":{\"headerSize\":26,\"margin\":15,\"minimumSpacing\":25,\"sides\":[{\"content\":{\"connectorIds\":[\"LConn1\"]},\"type\":\"ConnectorPlacement.EquallySpacedRectSide\",\"uuid\":\"315fc4b8-96c1-4575-a6b3-eadee3c565c5\"},{\"content\":{\"connectorIds\":[\"RConn1\"],\"side\":\"RIGHT\"},\"type\":\"ConnectorPlacement.EquallySpacedRectSide\",\"uuid\":\"3e876d4b-731c-46c4-97d4-16d95cf44eb6\"},{\"content\":{\"side\":\"TOP\"},\"type\":\"ConnectorPlacement.EquallySpacedRectSide\",\"uuid\":\"b527a8d5-4fb1-4a9d-8105-fff73624f75e\"}]},\"type\":\"ConnectorPlacement.EquallySpacedConnector\",\"uuid\":\"4da3c338-7f32-408f-a75b-02b41c006a8f\"}],\"packageUris\":[\"http://schema.mathworks.com/mf0/Connector/R2020b\"],\"version\":\"1.0\"}"
  Engine controller : Subsystem
      settings: PortSchema="{\"entries\":[{\"content\":{\"headerSize\":26,\"margin\":15,\"minimumSpacing\":25,\"sides\":[{\"content\":{\"connectorIds\":[\"LConn1\",\"In1\",\"In2\"]},\"type\":\"ConnectorPlacement.EquallySpacedRectSide\",\"uuid\":\"a24f90f9-b52e-4407-98a2-61cef3ed1001\"},{\"content\":{\"connectorIds\":[\"Out1\",\"Out2\",\"Out3\"],\"side\":\"RIGHT\"},\"type\":\"ConnectorPlacement.EquallySpacedRectSide\",\"uuid\":\"349c89d4-9966-4ad9-ba76-db4d38641e72\"},{\"content\":{\"side\":\"TOP\"},\"type\":\"ConnectorPlacement.EquallySpacedRectSide\",\"uuid\":\"c23b8a3e-5693-4bb4-96b3-90d999333c4e\"}]},\"type\":\"ConnectorPlacement.EquallySpacedConnector\",\"uuid\":\"ab682651-c32f-4460-8c4f-01dcf64563ad\"}],\"packageUris\":[\"http://schema.mathworks.com/mf0/Connector/R2020b\"],\"version\":\"1.0\"}"
  Ignition system : Subsystem
      settings: PortSchema="{\"entries\":[{\"content\":{\"headerSize\":26,\"margin\":15,\"minimumSpacing\":25,\"sides\":[{\"content\":{\"connectorIds\":[\"LConn1\"]},\"type\":\"ConnectorPlacement.EquallySpacedRectSide\",\"uuid\":\"a24f90f9-b52e-4407-98a2-61cef3ed1001\"},{\"content\":{\"connectorIds\":[\"RConn1\"],\"side\":\"RIGHT\"},\"type\":\"ConnectorPlacement.EquallySpacedRectSide\",\"uuid\":\"349c89d4-9966-4ad9-ba76-db4d38641e72\"},{\"content\":{\"side\":\"TOP\"},\"type\":\"ConnectorPlacement.EquallySpacedRectSide\",\"uuid\":\"c23b8a3e-5693-4bb4-96b3-90d999333c4e\"}]},\"type\":\"ConnectorPlacement.EquallySpacedConnector\",\"uuid\":\"ab682651-c32f-4460-8c4f-01dcf64563ad\"}],\"packageUris\":[\"http://schema.mathworks.com/mf0/Connector/R2020b\"],\"version\":\"1.0\"}"
  Mounting interface : Subsystem
      settings: PortSchema="{\"entries\":[{\"content\":{\"headerSize\":26,\"margin\":15,\"minimumSpacing\":25,\"sides\":[{\"content\":{\"connectorIds\":[\"LConn1\"]},\"type\":\"ConnectorPlacement.EquallySpacedRectSide\",\"uuid\":\"a24f90f9-b52e-4407-98a2-61cef3ed1001\"},{\"content\":{\"connectorIds\":[\"RConn1\"],\"side\":\"RIGHT\"},\"type\":\"ConnectorPlacement.EquallySpacedRectSide\",\"uuid\":\"349c89d4-9966-4ad9-ba76-db4d38641e72\"},{\"content\":{\"side\":\"TOP\"},\"type\":\"ConnectorPlacement.EquallySpacedRectSide\",\"uuid\":\"c23b8a3e-5693-4bb4-96b3-90d999333c4e\"}]},\"type\":\"ConnectorPlacement.EquallySpacedConnector\",\"uuid\":\"ab682651-c32f-4460-8c4f-01dcf64563ad\"}],\"packageUris\":[\"http://schema.mathworks.com/mf0/Connector/R2020b\"],\"version\":\"1.0\"}"
  Nozzle : Subsystem
      settings: PortSchema="{\"entries\":[{\"content\":{\"headerSize\":26,\"margin\":15,\"minimumSpacing\":25,\"sides\":[{\"content\":{\"connectorIds\":[\"LConn1\"]},\"type\":\"ConnectorPlacement.EquallySpacedRectSide\",\"uuid\":\"315fc4b8-96c1-4575-a6b3-eadee3c565c5\"},{\"content\":{\"connectorIds\":[\"Out1\"],\"side\":\"RIGHT\"},\"type\":\"ConnectorPlacement.EquallySpacedRectSide\",\"uuid\":\"3e876d4b-731c-46c4-97d4-16d95cf44eb6\"},{\"content\":{\"side\":\"TOP\"},\"type\":\"ConnectorPlacement.EquallySpacedRectSide\",\"uuid\":\"b527a8d5-4fb1-4a9d-8105-fff73624f75e\"}]},\"type\":\"ConnectorPlacement.EquallySpacedConnector\",\"uuid\":\"4da3c338-7f32-408f-a75b-02b41c006a8f\"}],\"packageUris\":[\"http://schema.mathworks.com/mf0/Connector/R2020b\"],\"version\":\"1.0\"}"
  Preburners : Subsystem
      settings: PortSchema="{\"entries\":[{\"content\":{\"headerSize\":26,\"margin\":15,\"minimumSpacing\":25,\"sides\":[{\"content\":{\"connectorIds\":[\"LConn1\",\"LConn2\"]},\"type\":\"ConnectorPlacement.EquallySpacedRectSide\",\"uuid\":\"315fc4b8-96c1-4575-a6b3-eadee3c565c5\"},{\"content\":{\"connectorIds\":[\"RConn1\"],\"side\":\"RIGHT\"},\"type\":\"ConnectorPlacement.EquallySpacedRectSide\",\"uuid\":\"3e876d4b-731c-46c4-97d4-16d95cf44eb6\"},{\"content\":{\"side\":\"TOP\"},\"type\":\"ConnectorPlacement.EquallySpacedRectSide\",\"uuid\":\"b527a8d5-4fb1-4a9d-8105-fff73624f75e\"}]},\"type\":\"ConnectorPlacement.EquallySpacedConnector\",\"uuid\":\"4da3c338-7f32-408f-a75b-02b41c006a8f\"}],\"packageUris\":[\"http://schema.mathworks.com/mf0/Connector/R2020b\"],\"version\":\"1.0\"}"
  Turbopumps : Subsystem
      settings: PortSchema="{\"entries\":[{\"content\":{\"headerSize\":26,\"margin\":15,\"minimumSpacing\":25,\"sides\":[{\"content\":{\"connectorIds\":[\"LConn1\",\"LConn2\"]},\"type\":\"ConnectorPlacement.EquallySpacedRectSide\",\"uuid\":\"315fc4b8-96c1-4575-a6b3-eadee3c565c5\"},{\"content\":{\"connectorIds\":[\"RConn1\",\"RConn2\"],\"side\":\"RIGHT\"},\"type\":\"ConnectorPlacement.EquallySpacedRectSide\",\"uuid\":\"3e876d4b-731c-46c4-97d4-16d95cf44eb6\"},{\"content\":{\"side\":\"TOP\"},\"type\":\"ConnectorPlacement.EquallySpacedRectSide\",\"uuid\":\"b527a8d5-4fb1-4a9d-8105-fff73624f75e\"}]},\"type\":\"ConnectorPlacement.EquallySpacedConnector\",\"uuid\":\"4da3c338-7f32-408f-a75b-02b41c006a8f\"}],\"packageUris\":[\"http://schema.mathworks.com/mf0/Connector/R2020b\"],\"version\":\"1.0\"}"
  Valves & control : Subsystem
      settings: PortSchema="{\"entries\":[{\"content\":{\"headerSize\":26,\"margin\":15,\"minimumSpacing\":25,\"sides\":[{\"content\":{\"connectorIds\":[\"In1\",\"LConn1\"]},\"type\":\"ConnectorPlacement.EquallySpacedRectSide\",\"uuid\":\"a24f90f9-b52e-4407-98a2-61cef3ed1001\"},{\"content\":{\"connectorIds\":[\"RConn1\"],\"side\":\"RIGHT\"},\"type\":\"ConnectorPlacement.EquallySpacedRectSide\",\"uuid\":\"349c89d4-9966-4ad9-ba76-db4d38641e72\"},{\"content\":{\"side\":\"TOP\"},\"type\":\"ConnectorPlacement.EquallySpacedRectSide\",\"uuid\":\"c23b8a3e-5693-4bb4-96b3-90d999333c4e\"}]},\"type\":\"ConnectorPlacement.EquallySpacedConnector\",\"uuid\":\"ab682651-c32f-4460-8c4f-01dcf64563ad\"}],\"packageUris\":[\"http://schema.mathworks.com/mf0/Connector/R2020b\"],\"version\":\"1.0\"}"
  IF-PWR-SEC-01 : PMIOPort  Side=Left  ConnectionType=Bus: ElectricalPower
  IF-SMT-TLI-01 : PMIOPort  Port=2  Side=Left  ConnectionType=Bus: StructuralLoad
  IF-SDM-STP-01 : PMIOPort  Port=3  Side=Left  ConnectionType=Bus: LiquidPropellantFeed
  IF-STP-SPR-01 : PMIOPort  Port=4  Side=Right  ConnectionType=Bus: AutogenousPressurantGas
  IF-SSG-SIG-01 : PMIOPort  Port=5  Side=Left  ConnectionType=Bus: SpinStartIgniterGas
  IF-SNG-SVC-01 : PMIOPort  Port=6  Side=Left  ConnectionType=Bus: PneumaticActuationGas
  IF-GMB-SMT-01 : PMIOPort  Port=7  Side=Left  ConnectionType=Bus: GimbalMotion
  Bus Element Out1 : Outport  PortName=IF-SEC-SAF-01
  Bus Element Out3 : Outport  Port=2  PortName=IF-SNZ-STP-01
  Bus Element Out2 : Outport  Port=3  PortName=IF-SEC-STA-01
  wires:
  Bus Element In2/1 -> Engine controller/2(IF-SAF-SEC-01)
  Bus Element In1/1 -> Engine controller/1(IF-GNC-SEC-01)
  Engine controller/3(IF-SEC-SVC-01) -> Valves & control/1(IF-SEC-SVC-01)
  Engine controller/2(IF-SEC-STA-01) -> Bus Element Out2/1
  Engine controller/1(IF-SEC-SAF-01) -> Bus Element Out1/1
  Nozzle/1(IF-SNZ-STP-01) -> Bus Element Out3/1
  connections:
  IF-SDM-STP-01/RConn1 -- Turbopumps/LConn1
  IF-GMB-SMT-01/RConn1 -- Mounting interface/LConn1
  Valves & control/RConn1 -- Turbopumps/LConn2
  Turbopumps/RConn2 -- Preburners/LConn1
  Ignition system/RConn1 -- Preburners/LConn2
  Preburners/RConn1 -- "Combustion Chamber "/LConn1
  "Combustion Chamber "/RConn1 -- Nozzle/LConn1
  IF-SSG-SIG-01/RConn1 -- Ignition system/LConn1
  IF-SNG-SVC-01/RConn1 -- Valves & control/LConn1
  Turbopumps/RConn1 -- IF-STP-SPR-01/RConn1
  IF-SMT-TLI-01/RConn1 -- Mounting interface/RConn1
  IF-PWR-SEC-01/RConn1 -- Engine controller/LConn1
